simulink model "fft_test"  (Simulink 7.4)
settings: Solver=VariableStepDiscrete  StartTime=0.0  StopTime=500  RelTol=1e-3
libraries: xbsIndex_r4 x1178, casper_library_misc x68, casper_library_delays x13, casper_library_reorder x4, casper_library_ffts_twiddle x2
(part 2 of 11)

== system fft_test/fft/fft_unscrambler ==
  sync : Inport  OutDataType=sfix(16)  OutScaling=2^0
  In1 : Inport  Port=2  OutDataType=sfix(16)  OutScaling=2^0
  In2 : Inport  Port=3  OutDataType=sfix(16)  OutScaling=2^0
  In3 : Inport  Port=4
  In4 : Inport  Port=5
  const : xbsIndex_r4/Constant  arith_type=Boolean  const=1  n_bits=1  bin_pt=0  explicit_period=on  period=1  equ=P=C  opselect=C  inp2=PCIN>>17  opr=+  inp1=P  carry=CIN  dbl_ovrd=off  block_type=constant
      settings: block_version=9.1.01
  reorder : Subsystem  AncestorBlock=casper_library_reorder/reorder  mask(reorder){map=getfield( getfield( get_param( gcb,'UserData' ), 'parameters'),'map'), n_inputs=4, bram_latency=1, map_latency=1, double_buffer=0}
      mask prompts: map "Output Order:"; n_inputs "Number of inputs"; bram_latency "BRAM Latency"; map_latency "Map Latency"; double_buffer "Double Buffer"
      mask init:
      | reorder_init(gcb, ...
      |     'map', map, ...
      |     'n_inputs', n_inputs, ...
      |     'bram_latency', bram_latency, ...
      |     'map_latency', map_latency, ...
      |     'double_buffer', double_buffer);
      settings: AttributesFormatString=order=2
  square_transposer : Subsystem  AncestorBlock=casper_library_reorder/square_transposer  mask(square_transposer){n_inputs=2}
      mask prompts: n_inputs "Number of inputs (2^?):"
      mask init:
      | square_transposer_init(gcb,...
      |     'n_inputs', n_inputs);
      settings: AttributesFormatString=n_inputs=2
  sync_out : Outport  OutDataType=sfix(16)  OutScaling=2^0
  Out1 : Outport  Port=2  OutDataType=sfix(16)  OutScaling=2^0
  Out2 : Outport  Port=3  OutDataType=sfix(16)  OutScaling=2^0
  Out3 : Outport  Port=4
  Out4 : Outport  Port=5
  wires:
  sync/1 -> square_transposer/1(sync)
  square_transposer/1(sync_out) -> reorder/1(sync)
  reorder/1(sync_out) -> sync_out/1
  const/1 -> reorder/2(en)
  In1/1 -> square_transposer/2(In1)
  square_transposer/2(Out1) -> reorder/3(din0)
  reorder/3(dout0) -> Out1/1
  In2/1 -> square_transposer/3(In2)
  square_transposer/3(Out2) -> reorder/4(din1)
  reorder/4(dout1) -> Out2/1
  In3/1 -> square_transposer/4(In3)
  square_transposer/4(Out3) -> reorder/5(din2)
  reorder/5(dout2) -> Out3/1
  In4/1 -> square_transposer/5(In4)
  square_transposer/5(Out4) -> reorder/6(din3)
  reorder/6(dout3) -> Out4/1

== system fft_test/fft/fft_biplex0/biplex_core ==
  pol1 : Inport
  pol2 : Inport  Port=2
  sync : Inport  Port=3
  shift : Inport  Port=4
  Constant : xbsIndex_r4/Constant  arith_type=Boolean  const=0  n_bits=16  bin_pt=14  explicit_period=off  period=1  equ=P=C  opselect=C  inp2=PCIN>>17  opr=+  inp1=P  carry=CIN  dbl_ovrd=off  block_type=constant
      settings: block_version=11.4
  fft_stage_1 : Subsystem  AncestorBlock=casper_library_ffts/fft_stage_n  mask(fft_stage_n){FFTSize=4, FFTStage=1, input_bit_width=8, coeff_bit_width=8, delays_bram=off, coeffs_bram=off, quantization=Round  (unbiased: +/- Inf), overflow=Saturate, add_latency=2, mult_latency=3, bram_latency=1, conv_latency=2, arch=Virtex5, opt_target=multipliers, use_hdl=on, use_embedded=off, dsp48_adders=on}
      mask prompts: FFTSize "Size of FFT: (2^? pnts)"; FFTStage "Stage of FFT:"; input_bit_width "Input/Output Bit Width:"; coeff_bit_width "Coefficient Bit Width"; delays_bram "Implement Delays in BRAM:"; coeffs_bram "Store Coefficients in BRAM:"; quantization "Quantization Behavior"; overflow "Overflow Behavior"; add_latency "Add Latency"; mult_latency "Mult Latency"; bram_latency "BRAM Latency"; conv_latency "Convert latency"; arch "Architecture"; opt_target "Use less"; use_hdl "Use behavioural HDL for mutlipliers"; use_embedded "Use embedded multipliers"; dsp48_adders "Use DSP48s for adders"
      mask init:
      | fft_stage_n_init(gcb,...
      |     'FFTSize', FFTSize,...
      |     'FFTStage', FFTStage,...
      |     'input_bit_width', input_bit_width,...
      |     'coeff_bit_width', coeff_bit_width,...
      |     'delays_bram', delays_bram,...
      |     'coeffs_bram', coeffs_bram,...
      |     'quantization', quantization,...
      |     'overflow', overflow,...
      |     'add_latency', add_latency,...
      |     'mult_latency', mult_latency,...
      |     'bram_latency', bram_latency,...
      |     'conv_latency', conv_latency, ...
      |     'arch', arch, ...
      |     'opt_target', opt_target, ...
      |     'use_hdl', use_hdl,...
      |     'use_embedded', use_embedded, ...
      |     'dsp48_adders', dsp48_adders);
      settings: AttributesFormatString=|
      | [1/4]
      | delays in slices
      | coeffs in slices
      mask StyleString: edit,edit,edit,edit,checkbox,checkbox,popup(Truncate|Round  (unbiased: +/- Inf)|Round  (unbiased: Even Values)),popup(Wrap|Saturate|Error),edit,edit,edit,edit,popup(Virtex2Pro|Virtex5),popup(logic|multipliers),checkbox,checkbox,checkbox
      mask CallbackString:
      | ||||||||||||fft_callback_arch(gcb);||use_hdl = get_param(gcb,'use_hdl');
      | visibs = get_param(gcb, 'MaskVisibilities');
      | if( strcmp(use_hdl,'on')),
      |     visibs{16} = 'off';
      | else,
      |     visibs{16} = 'on';
      | end
      |     set_param(gcb, 'MaskVisibilities',visibs);||fft_callback_dsp48_adders(gcb);
  fft_stage_2 : Subsystem  AncestorBlock=casper_library_ffts/fft_stage_n  mask(fft_stage_n){FFTSize=4, FFTStage=2, input_bit_width=8, coeff_bit_width=8, delays_bram=off, coeffs_bram=off, quantization=Round  (unbiased: +/- Inf), overflow=Saturate, add_latency=2, mult_latency=3, bram_latency=1, conv_latency=2, arch=Virtex5, opt_target=multipliers, use_hdl=off, use_embedded=on, dsp48_adders=on}
      mask prompts: FFTSize "Size of FFT: (2^? pnts)"; FFTStage "Stage of FFT:"; input_bit_width "Input/Output Bit Width:"; coeff_bit_width "Coefficient Bit Width"; delays_bram "Implement Delays in BRAM:"; coeffs_bram "Store Coefficients in BRAM:"; quantization "Quantization Behavior"; overflow "Overflow Behavior"; add_latency "Add Latency"; mult_latency "Mult Latency"; bram_latency "BRAM Latency"; conv_latency "Convert latency"; arch "Architecture"; opt_target "Use less"; use_hdl "Use behavioural HDL for mutlipliers"; use_embedded "Use embedded multipliers"; dsp48_adders "Use DSP48s for adders"
      mask init: same as fft_test/fft/fft_biplex0/biplex_core/fft_stage_1
      settings: AttributesFormatString=|
      | [2/4]
      | delays in slices
      | coeffs in slices
      mask StyleString: edit,edit,edit,edit,checkbox,checkbox,popup(Truncate|Round  (unbiased: +/- Inf)|Round  (unbiased: Even Values)),popup(Wrap|Saturate|Error),edit,edit,edit,edit,popup(Virtex2Pro|Virtex5),popup(logic|multipliers),checkbox,checkbox,checkbox
      mask CallbackString:
      | ||||||||||||fft_callback_arch(gcb);||use_hdl = get_param(gcb,'use_hdl');
      | visibs = get_param(gcb, 'MaskVisibilities');
      | if( strcmp(use_hdl,'on')),
      |     visibs{16} = 'off';
      | else,
      |     visibs{16} = 'on';
      | end
      |     set_param(gcb, 'MaskVisibilities',visibs);||fft_callback_dsp48_adders(gcb);
  fft_stage_3 : Subsystem  AncestorBlock=casper_library_ffts/fft_stage_n  mask(fft_stage_n){FFTSize=4, FFTStage=3, input_bit_width=8, coeff_bit_width=8, delays_bram=off, coeffs_bram=off, quantization=Round  (unbiased: +/- Inf), overflow=Saturate, add_latency=2, mult_latency=3, bram_latency=1, conv_latency=2, arch=Virtex5, opt_target=multipliers, use_hdl=on, use_embedded=off, dsp48_adders=on}
      mask prompts: FFTSize "Size of FFT: (2^? pnts)"; FFTStage "Stage of FFT:"; input_bit_width "Input/Output Bit Width:"; coeff_bit_width "Coefficient Bit Width"; delays_bram "Implement Delays in BRAM:"; coeffs_bram "Store Coefficients in BRAM:"; quantization "Quantization Behavior"; overflow "Overflow Behavior"; add_latency "Add Latency"; mult_latency "Mult Latency"; bram_latency "BRAM Latency"; conv_latency "Convert latency"; arch "Architecture"; opt_target "Use less"; use_hdl "Use behavioural HDL for mutlipliers"; use_embedded "Use embedded multipliers"; dsp48_adders "Use DSP48s for adders"
      mask init: same as fft_test/fft/fft_biplex0/biplex_core/fft_stage_1
      settings: AttributesFormatString=|
      | [3/4]
      | delays in slices
      | coeffs in slices
      mask StyleString: edit,edit,edit,edit,checkbox,checkbox,popup(Truncate|Round  (unbiased: +/- Inf)|Round  (unbiased: Even Values)),popup(Wrap|Saturate|Error),edit,edit,edit,edit,popup(Virtex2Pro|Virtex5),popup(logic|multipliers),checkbox,checkbox,checkbox
      mask CallbackString:
      | ||||||||||||fft_callback_arch(gcb);||use_hdl = get_param(gcb,'use_hdl');
      | visibs = get_param(gcb, 'MaskVisibilities');
      | if( strcmp(use_hdl,'on')),
      |     visibs{16} = 'off';
      | else,
      |     visibs{16} = 'on';
      | end
      |     set_param(gcb, 'MaskVisibilities',visibs);||fft_callback_dsp48_adders(gcb);
  fft_stage_4 : Subsystem  AncestorBlock=casper_library_ffts/fft_stage_n  mask(fft_stage_n){FFTSize=4, FFTStage=4, input_bit_width=8, coeff_bit_width=8, delays_bram=off, coeffs_bram=off, quantization=Round  (unbiased: +/- Inf), overflow=Saturate, add_latency=2, mult_latency=3, bram_latency=1, conv_latency=2, arch=Virtex5, opt_target=multipliers, use_hdl=on, use_embedded=off, dsp48_adders=on}
      mask prompts: FFTSize "Size of FFT: (2^? pnts)"; FFTStage "Stage of FFT:"; input_bit_width "Input/Output Bit Width:"; coeff_bit_width "Coefficient Bit Width"; delays_bram "Implement Delays in BRAM:"; coeffs_bram "Store Coefficients in BRAM:"; quantization "Quantization Behavior"; overflow "Overflow Behavior"; add_latency "Add Latency"; mult_latency "Mult Latency"; bram_latency "BRAM Latency"; conv_latency "Convert latency"; arch "Architecture"; opt_target "Use less"; use_hdl "Use behavioural HDL for mutlipliers"; use_embedded "Use embedded multipliers"; dsp48_adders "Use DSP48s for adders"
      mask init: same as fft_test/fft/fft_biplex0/biplex_core/fft_stage_1
      settings: AttributesFormatString=|
      | [4/4]
      | delays in slices
      | coeffs in slices
      mask StyleString: edit,edit,edit,edit,checkbox,checkbox,popup(Truncate|Round  (unbiased: +/- Inf)|Round  (unbiased: Even Values)),popup(Wrap|Saturate|Error),edit,edit,edit,edit,popup(Virtex2Pro|Virtex5),popup(logic|multipliers),checkbox,checkbox,checkbox
      mask CallbackString:
      | ||||||||||||fft_callback_arch(gcb);||use_hdl = get_param(gcb,'use_hdl');
      | visibs = get_param(gcb, 'MaskVisibilities');
      | if( strcmp(use_hdl,'on')),
      |     visibs{16} = 'off';
      | else,
      |     visibs{16} = 'on';
      | end
      |     set_param(gcb, 'MaskVisibilities',visibs);||fft_callback_dsp48_adders(gcb);
  out1 : Outport
  out2 : Outport  Port=2
  of : Outport  Port=3
  sync_out : Outport  Port=4
  wires:
  fft_stage_1/1(out1) -> fft_stage_2/1(in1)
  fft_stage_1/2(out2) -> fft_stage_2/2(in2)
  fft_stage_1/3(of) -> fft_stage_2/3(of_in)
  fft_stage_1/4(sync_out) -> fft_stage_2/4(sync)
  shift/1 -> fft_stage_2/5(shift), fft_stage_3/5(shift), fft_stage_4/5(shift), fft_stage_1/5(shift)
  fft_stage_2/1(out1) -> fft_stage_3/1(in1)
  fft_stage_2/2(out2) -> fft_stage_3/2(in2)
  fft_stage_2/3(of) -> fft_stage_3/3(of_in)
  fft_stage_2/4(sync_out) -> fft_stage_3/4(sync)
  fft_stage_3/1(out1) -> fft_stage_4/1(in1)
  fft_stage_3/2(out2) -> fft_stage_4/2(in2)
  fft_stage_3/3(of) -> fft_stage_4/3(of_in)
  fft_stage_3/4(sync_out) -> fft_stage_4/4(sync)
  pol1/1 -> fft_stage_1/1(in1)
  pol2/1 -> fft_stage_1/2(in2)
  Constant/1 -> fft_stage_1/3(of_in)
  sync/1 -> fft_stage_1/4(sync)
  fft_stage_4/1(out1) -> out1/1
  fft_stage_4/2(out2) -> out2/1
  fft_stage_4/3(of) -> of/1
  fft_stage_4/4(sync_out) -> sync_out/1

== system fft_test/fft/fft_biplex0/biplex_cplx_unscrambler ==
  even : Inport  OutDataType=sfix(16)  OutScaling=2^0
  odd : Inport  Port=2  OutDataType=sfix(16)  OutScaling=2^0
  sync : Inport  Port=3  OutDataType=sfix(16)  OutScaling=2^0
  Constant : xbsIndex_r4/Constant  arith_type=Boolean  const=1  n_bits=1  bin_pt=0  explicit_period=on  period=1  equ=P=C  opselect=C  inp2=PCIN>>17  opr=+  inp1=P  carry=CIN  dbl_ovrd=off  block_type=constant
      settings: block_version=9.1.01
  Constant1 : xbsIndex_r4/Constant  arith_type=Unsigned  const=2^(FFTSize-1)  n_bits=FFTSize  bin_pt=0  explicit_period=on  period=1  equ=P=C  opselect=C  inp2=PCIN>>17  opr=+  inp1=P  carry=CIN  dbl_ovrd=off  block_type=constant
      settings: block_version=9.1.01
  Constant2 : xbsIndex_r4/Constant  arith_type=Unsigned  const=2^(FFTSize-1)  n_bits=FFTSize  bin_pt=0  explicit_period=on  period=1  equ=P=C  opselect=C  inp2=PCIN>>17  opr=+  inp1=P  carry=CIN  dbl_ovrd=off  block_type=constant
      settings: block_version=9.1.01
  Convert : xbsIndex_r4/Convert  arith_type=Unsigned  n_bits=1  bin_pt=0  quantization=Truncate  overflow=Wrap  latency=0  dbl_ovrd=off  pipeline=off  block_type=convert
      settings: xl_area=[0, 0, 0, 0, 0, 0, 0]
  Convert1 : xbsIndex_r4/Convert  arith_type=Unsigned  n_bits=1  bin_pt=0  quantization=Truncate  overflow=Wrap  latency=0  dbl_ovrd=off  pipeline=off  block_type=convert
      settings: xl_area=[0, 0, 0, 0, 0, 0, 0]
  Counter : xbsIndex_r4/Counter  cnt_type=Free Running  cnt_to=Inf  operation=Up  start_count=0  cnt_by_val=1  arith_type=Unsigned  n_bits=FFTSize  bin_pt=0  load_pin=off  rst=on  en=off  explicit_period=off  period=1  dbl_ovrd=off  use_behavioral_HDL=off  implementation=Fabric  use_rpm=on  block_type=counter
      settings: xl_area=[0, 0, 0, 0, 0, 0, 0]  block_version=9.1.01
  Counter1 : xbsIndex_r4/Counter  cnt_type=Free Running  cnt_to=Inf  operation=Up  start_count=0  cnt_by_val=1  arith_type=Unsigned  n_bits=FFTSize  bin_pt=0  load_pin=off  rst=on  en=off  explicit_period=off  period=1  dbl_ovrd=off  use_behavioral_HDL=off  implementation=Fabric  use_rpm=on  block_type=counter
      settings: xl_area=[0, 0, 0, 0, 0, 0, 0]  block_version=9.1.01
  Relational : xbsIndex_r4/Relational  mode=a<=b  en=off  latency=0  dbl_ovrd=off  block_type=relational
      settings: xl_area=[0, 0, 0, 0, 0, 0, 0]  block_version=9.1.01
  Relational1 : xbsIndex_r4/Relational  mode=a<=b  en=off  latency=0  dbl_ovrd=off  block_type=relational
      settings: xl_area=[0, 0, 0, 0, 0, 0, 0]  block_version=9.1.01
  barrel_switcher : casper_library_reorder/barrel_switcher  SystemSampleTime=-1  n_inputs=1
      settings: AttributesFormatString=n_inputs=1
  barrel_switcher1 : casper_library_reorder/barrel_switcher  SystemSampleTime=-1  n_inputs=1
      settings: AttributesFormatString=n_inputs=1
  reorder : Subsystem  AncestorBlock=casper_library_reorder/reorder  mask(reorder){map=getfield( getfield( get_param( gcb,'UserData' ), 'parameters'),'map'), n_inputs=1, bram_latency=1, map_latency=0, double_buffer=0, bram_map=off}
      mask prompts: map "Output Order:"; n_inputs "Number of inputs"; bram_latency "BRAM Latency"; map_latency "Map Latency"; double_buffer "Double Buffer"; bram_map "Use BlockRAM for Map"
      mask init:
      | reorder_init(gcb, ...
      |     'map', map, ...
      |     'n_inputs', n_inputs, ...
      |     'bram_latency', bram_latency, ...
      |     'map_latency', map_latency, ...
      |     'double_buffer', double_buffer, ...
      |     'bram_map', bram_map);
      settings: AttributesFormatString=order=2
      mask Help: eval('xlWeb(''http://casper.berkeley.edu/wiki/Reorder'')')
  reorder1 : Subsystem  AncestorBlock=casper_library_reorder/reorder  mask(reorder){map=getfield( getfield( get_param( gcb,'UserData' ), 'parameters'),'map'), n_inputs=1, bram_latency=1, map_latency=0, double_buffer=0, bram_map=off}
      mask prompts: map "Output Order:"; n_inputs "Number of inputs"; bram_latency "BRAM Latency"; map_latency "Map Latency"; double_buffer "Double Buffer"; bram_map "Use BlockRAM for Map"
      mask init: same as fft_test/fft/fft_biplex0/biplex_cplx_unscrambler/reorder
      settings: AttributesFormatString=order=2
      mask Help: eval('xlWeb(''http://casper.berkeley.edu/wiki/Reorder'')')
  pol1 : Outport  OutDataType=sfix(16)  OutScaling=2^0
  pol2 : Outport  Port=2  OutDataType=sfix(16)  OutScaling=2^0
  sync_out : Outport  Port=3  OutDataType=sfix(16)  OutScaling=2^0
  wires:
  barrel_switcher/1 -> reorder/1(sync), reorder1/1(sync)
  barrel_switcher/2 -> reorder/3(din0)
  barrel_switcher/3 -> reorder1/3(din0)
  reorder/1(sync_out) -> barrel_switcher1/2, Counter1/1
  reorder/3(dout0) -> barrel_switcher1/3
  reorder1/3(dout0) -> barrel_switcher1/4
  even/1 -> barrel_switcher/3
  odd/1 -> barrel_switcher/4
  barrel_switcher1/1 -> sync_out/1
  barrel_switcher1/2 -> pol1/1
  barrel_switcher1/3 -> pol2/1
  sync/1 -> barrel_switcher/2, Counter/1
  Constant/1 -> reorder/2(en), reorder1/2(en)
  Constant1/1 -> Relational/1
  Counter/1 -> Relational/2
  Counter1/1 -> Relational1/2
  Constant2/1 -> Relational1/1
  Relational/1 -> Convert/1
  Relational1/1 -> Convert1/1
  Convert1/1 -> barrel_switcher1/1
  Convert/1 -> barrel_switcher/1

== system fft_test/fft/fft_biplex1/biplex_core ==
  pol1 : Inport
  pol2 : Inport  Port=2
  sync : Inport  Port=3
  shift : Inport  Port=4
  Constant : xbsIndex_r4/Constant  arith_type=Boolean  const=0  n_bits=16  bin_pt=14  explicit_period=off  period=1  equ=P=C  opselect=C  inp2=PCIN>>17  opr=+  inp1=P  carry=CIN  dbl_ovrd=off  block_type=constant
      settings: block_version=11.4
  fft_stage_1 : Subsystem  AncestorBlock=casper_library_ffts/fft_stage_n  mask(fft_stage_n){FFTSize=4, FFTStage=1, input_bit_width=8, coeff_bit_width=8, delays_bram=off, coeffs_bram=off, quantization=Round  (unbiased: +/- Inf), overflow=Saturate, add_latency=2, mult_latency=3, bram_latency=1, conv_latency=2, arch=Virtex5, opt_target=multipliers, use_hdl=on, use_embedded=off, dsp48_adders=on}
      mask prompts: FFTSize "Size of FFT: (2^? pnts)"; FFTStage "Stage of FFT:"; input_bit_width "Input/Output Bit Width:"; coeff_bit_width "Coefficient Bit Width"; delays_bram "Implement Delays in BRAM:"; coeffs_bram "Store Coefficients in BRAM:"; quantization "Quantization Behavior"; overflow "Overflow Behavior"; add_latency "Add Latency"; mult_latency "Mult Latency"; bram_latency "BRAM Latency"; conv_latency "Convert latency"; arch "Architecture"; opt_target "Use less"; use_hdl "Use behavioural HDL for mutlipliers"; use_embedded "Use embedded multipliers"; dsp48_adders "Use DSP48s for adders"
      mask init: same as fft_test/fft/fft_biplex0/biplex_core/fft_stage_1
      settings: AttributesFormatString=|
      | [1/4]
      | delays in slices
      | coeffs in slices
      mask StyleString: edit,edit,edit,edit,checkbox,checkbox,popup(Truncate|Round  (unbiased: +/- Inf)|Round  (unbiased: Even Values)),popup(Wrap|Saturate|Error),edit,edit,edit,edit,popup(Virtex2Pro|Virtex5),popup(logic|multipliers),checkbox,checkbox,checkbox
      mask CallbackString:
      | ||||||||||||fft_callback_arch(gcb);||use_hdl = get_param(gcb,'use_hdl');
      | visibs = get_param(gcb, 'MaskVisibilities');
      | if( strcmp(use_hdl,'on')),
      |     visibs{16} = 'off';
      | else,
      |     visibs{16} = 'on';
      | end
      |     set_param(gcb, 'MaskVisibilities',visibs);||fft_callback_dsp48_adders(gcb);
  fft_stage_2 : Subsystem  AncestorBlock=casper_library_ffts/fft_stage_n  mask(fft_stage_n){FFTSize=4, FFTStage=2, input_bit_width=8, coeff_bit_width=8, delays_bram=off, coeffs_bram=off, quantization=Round  (unbiased: +/- Inf), overflow=Saturate, add_latency=2, mult_latency=3, bram_latency=1, conv_latency=2, arch=Virtex5, opt_target=multipliers, use_hdl=off, use_embedded=on, dsp48_adders=on}
      mask prompts: FFTSize "Size of FFT: (2^? pnts)"; FFTStage "Stage of FFT:"; input_bit_width "Input/Output Bit Width:"; coeff_bit_width "Coefficient Bit Width"; delays_bram "Implement Delays in BRAM:"; coeffs_bram "Store Coefficients in BRAM:"; quantization "Quantization Behavior"; overflow "Overflow Behavior"; add_latency "Add Latency"; mult_latency "Mult Latency"; bram_latency "BRAM Latency"; conv_latency "Convert latency"; arch "Architecture"; opt_target "Use less"; use_hdl "Use behavioural HDL for mutlipliers"; use_embedded "Use embedded multipliers"; dsp48_adders "Use DSP48s for adders"
      mask init: same as fft_test/fft/fft_biplex0/biplex_core/fft_stage_1
      settings: AttributesFormatString=|
      | [2/4]
      | delays in slices
      | coeffs in slices
      mask StyleString: edit,edit,edit,edit,checkbox,checkbox,popup(Truncate|Round  (unbiased: +/- Inf)|Round  (unbiased: Even Values)),popup(Wrap|Saturate|Error),edit,edit,edit,edit,popup(Virtex2Pro|Virtex5),popup(logic|multipliers),checkbox,checkbox,checkbox
      mask CallbackString:
      | ||||||||||||fft_callback_arch(gcb);||use_hdl = get_param(gcb,'use_hdl');
      | visibs = get_param(gcb, 'MaskVisibilities');
      | if( strcmp(use_hdl,'on')),
      |     visibs{16} = 'off';
      | else,
      |     visibs{16} = 'on';
      | end
      |     set_param(gcb, 'MaskVisibilities',visibs);||fft_callback_dsp48_adders(gcb);
  fft_stage_3 : Subsystem  AncestorBlock=casper_library_ffts/fft_stage_n  mask(fft_stage_n){FFTSize=4, FFTStage=3, input_bit_width=8, coeff_bit_width=8, delays_bram=off, coeffs_bram=off, quantization=Round  (unbiased: +/- Inf), overflow=Saturate, add_latency=2, mult_latency=3, bram_latency=1, conv_latency=2, arch=Virtex5, opt_target=multipliers, use_hdl=on, use_embedded=off, dsp48_adders=on}
      mask prompts: FFTSize "Size of FFT: (2^? pnts)"; FFTStage "Stage of FFT:"; input_bit_width "Input/Output Bit Width:"; coeff_bit_width "Coefficient Bit Width"; delays_bram "Implement Delays in BRAM:"; coeffs_bram "Store Coefficients in BRAM:"; quantization "Quantization Behavior"; overflow "Overflow Behavior"; add_latency "Add Latency"; mult_latency "Mult Latency"; bram_latency "BRAM Latency"; conv_latency "Convert latency"; arch "Architecture"; opt_target "Use less"; use_hdl "Use behavioural HDL for mutlipliers"; use_embedded "Use embedded multipliers"; dsp48_adders "Use DSP48s for adders"
      mask init: same as fft_test/fft/fft_biplex0/biplex_core/fft_stage_1
      settings: AttributesFormatString=|
      | [3/4]
      | delays in slices
      | coeffs in slices
      mask StyleString: edit,edit,edit,edit,checkbox,checkbox,popup(Truncate|Round  (unbiased: +/- Inf)|Round  (unbiased: Even Values)),popup(Wrap|Saturate|Error),edit,edit,edit,edit,popup(Virtex2Pro|Virtex5),popup(logic|multipliers),checkbox,checkbox,checkbox
      mask CallbackString:
      | ||||||||||||fft_callback_arch(gcb);||use_hdl = get_param(gcb,'use_hdl');
      | visibs = get_param(gcb, 'MaskVisibilities');
      | if( strcmp(use_hdl,'on')),
      |     visibs{16} = 'off';
      | else,
      |     visibs{16} = 'on';
      | end
      |     set_param(gcb, 'MaskVisibilities',visibs);||fft_callback_dsp48_adders(gcb);
  fft_stage_4 : Subsystem  AncestorBlock=casper_library_ffts/fft_stage_n  mask(fft_stage_n){FFTSize=4, FFTStage=4, input_bit_width=8, coeff_bit_width=8, delays_bram=off, coeffs_bram=off, quantization=Round  (unbiased: +/- Inf), overflow=Saturate, add_latency=2, mult_latency=3, bram_latency=1, conv_latency=2, arch=Virtex5, opt_target=multipliers, use_hdl=on, use_embedded=off, dsp48_adders=on}
      mask prompts: FFTSize "Size of FFT: (2^? pnts)"; FFTStage "Stage of FFT:"; input_bit_width "Input/Output Bit Width:"; coeff_bit_width "Coefficient Bit Width"; delays_bram "Implement Delays in BRAM:"; coeffs_bram "Store Coefficients in BRAM:"; quantization "Quantization Behavior"; overflow "Overflow Behavior"; add_latency "Add Latency"; mult_latency "Mult Latency"; bram_latency "BRAM Latency"; conv_latency "Convert latency"; arch "Architecture"; opt_target "Use less"; use_hdl "Use behavioural HDL for mutlipliers"; use_embedded "Use embedded multipliers"; dsp48_adders "Use DSP48s for adders"
      mask init: same as fft_test/fft/fft_biplex0/biplex_core/fft_stage_1
      settings: AttributesFormatString=|
      | [4/4]
      | delays in slices
      | coeffs in slices
      mask StyleString: edit,edit,edit,edit,checkbox,checkbox,popup(Truncate|Round  (unbiased: +/- Inf)|Round  (unbiased: Even Values)),popup(Wrap|Saturate|Error),edit,edit,edit,edit,popup(Virtex2Pro|Virtex5),popup(logic|multipliers),checkbox,checkbox,checkbox
      mask CallbackString:
      | ||||||||||||fft_callback_arch(gcb);||use_hdl = get_param(gcb,'use_hdl');
      | visibs = get_param(gcb, 'MaskVisibilities');
      | if( strcmp(use_hdl,'on')),
      |     visibs{16} = 'off';
      | else,
      |     visibs{16} = 'on';
      | end
      |     set_param(gcb, 'MaskVisibilities',visibs);||fft_callback_dsp48_adders(gcb);
  out1 : Outport
  out2 : Outport  Port=2
  of : Outport  Port=3
  sync_out : Outport  Port=4
  wires:
  fft_stage_1/1(out1) -> fft_stage_2/1(in1)
  fft_stage_1/2(out2) -> fft_stage_2/2(in2)
  fft_stage_1/3(of) -> fft_stage_2/3(of_in)
  fft_stage_1/4(sync_out) -> fft_stage_2/4(sync)
  shift/1 -> fft_stage_2/5(shift), fft_stage_3/5(shift), fft_stage_4/5(shift), fft_stage_1/5(shift)
  fft_stage_2/1(out1) -> fft_stage_3/1(in1)
  fft_stage_2/2(out2) -> fft_stage_3/2(in2)
  fft_stage_2/3(of) -> fft_stage_3/3(of_in)
  fft_stage_2/4(sync_out) -> fft_stage_3/4(sync)
  fft_stage_3/1(out1) -> fft_stage_4/1(in1)
  fft_stage_3/2(out2) -> fft_stage_4/2(in2)
  fft_stage_3/3(of) -> fft_stage_4/3(of_in)
  fft_stage_3/4(sync_out) -> fft_stage_4/4(sync)
  pol1/1 -> fft_stage_1/1(in1)
  pol2/1 -> fft_stage_1/2(in2)
  Constant/1 -> fft_stage_1/3(of_in)
  sync/1 -> fft_stage_1/4(sync)
  fft_stage_4/1(out1) -> out1/1
  fft_stage_4/2(out2) -> out2/1
  fft_stage_4/3(of) -> of/1
  fft_stage_4/4(sync_out) -> sync_out/1

== system fft_test/fft/fft_biplex1/biplex_cplx_unscrambler ==
  even : Inport  OutDataType=sfix(16)  OutScaling=2^0
  odd : Inport  Port=2  OutDataType=sfix(16)  OutScaling=2^0
  sync : Inport  Port=3  OutDataType=sfix(16)  OutScaling=2^0
  Constant : xbsIndex_r4/Constant  arith_type=Boolean  const=1  n_bits=1  bin_pt=0  explicit_period=on  period=1  equ=P=C  opselect=C  inp2=PCIN>>17  opr=+  inp1=P  carry=CIN  dbl_ovrd=off  block_type=constant
      settings: block_version=9.1.01
  Constant1 : xbsIndex_r4/Constant  arith_type=Unsigned  const=2^(FFTSize-1)  n_bits=FFTSize  bin_pt=0  explicit_period=on  period=1  equ=P=C  opselect=C  inp2=PCIN>>17  opr=+  inp1=P  carry=CIN  dbl_ovrd=off  block_type=constant
      settings: block_version=9.1.01
  Constant2 : xbsIndex_r4/Constant  arith_type=Unsigned  const=2^(FFTSize-1)  n_bits=FFTSize  bin_pt=0  explicit_period=on  period=1  equ=P=C  opselect=C  inp2=PCIN>>17  opr=+  inp1=P  carry=CIN  dbl_ovrd=off  block_type=constant
      settings: block_version=9.1.01
  Convert : xbsIndex_r4/Convert  arith_type=Unsigned  n_bits=1  bin_pt=0  quantization=Truncate  overflow=Wrap  latency=0  dbl_ovrd=off  pipeline=off  block_type=convert
      settings: xl_area=[0, 0, 0, 0, 0, 0, 0]
  Convert1 : xbsIndex_r4/Convert  arith_type=Unsigned  n_bits=1  bin_pt=0  quantization=Truncate  overflow=Wrap  latency=0  dbl_ovrd=off  pipeline=off  block_type=convert
      settings: xl_area=[0, 0, 0, 0, 0, 0, 0]
  Counter : xbsIndex_r4/Counter  cnt_type=Free Running  cnt_to=Inf  operation=Up  start_count=0  cnt_by_val=1  arith_type=Unsigned  n_bits=FFTSize  bin_pt=0  load_pin=off  rst=on  en=off  explicit_period=off  period=1  dbl_ovrd=off  use_behavioral_HDL=off  implementation=Fabric  use_rpm=on  block_type=counter
      settings: xl_area=[0, 0, 0, 0, 0, 0, 0]  block_version=9.1.01
  Counter1 : xbsIndex_r4/Counter  cnt_type=Free Running  cnt_to=Inf  operation=Up  start_count=0  cnt_by_val=1  arith_type=Unsigned  n_bits=FFTSize  bin_pt=0  load_pin=off  rst=on  en=off  explicit_period=off  period=1  dbl_ovrd=off  use_behavioral_HDL=off  implementation=Fabric  use_rpm=on  block_type=counter
      settings: xl_area=[0, 0, 0, 0, 0, 0, 0]  block_version=9.1.01
  Relational : xbsIndex_r4/Relational  mode=a<=b  en=off  latency=0  dbl_ovrd=off  block_type=relational
      settings: xl_area=[0, 0, 0, 0, 0, 0, 0]  block_version=9.1.01
  Relational1 : xbsIndex_r4/Relational  mode=a<=b  en=off  latency=0  dbl_ovrd=off  block_type=relational
      settings: xl_area=[0, 0, 0, 0, 0, 0, 0]  block_version=9.1.01
  barrel_switcher : casper_library_reorder/barrel_switcher  SystemSampleTime=-1  n_inputs=1
      settings: AttributesFormatString=n_inputs=1
  barrel_switcher1 : casper_library_reorder/barrel_switcher  SystemSampleTime=-1  n_inputs=1
      settings: AttributesFormatString=n_inputs=1
  reorder : Subsystem  AncestorBlock=casper_library_reorder/reorder  mask(reorder){map=getfield( getfield( get_param( gcb,'UserData' ), 'parameters'),'map'), n_inputs=1, bram_latency=1, map_latency=0, double_buffer=0, bram_map=off}
      mask prompts: map "Output Order:"; n_inputs "Number of inputs"; bram_latency "BRAM Latency"; map_latency "Map Latency"; double_buffer "Double Buffer"; bram_map "Use BlockRAM for Map"
      mask init: same as fft_test/fft/fft_biplex0/biplex_cplx_unscrambler/reorder
      settings: AttributesFormatString=order=2
      mask Help: eval('xlWeb(''http://casper.berkeley.edu/wiki/Reorder'')')
  reorder1 : Subsystem  AncestorBlock=casper_library_reorder/reorder  mask(reorder){map=getfield( getfield( get_param( gcb,'UserData' ), 'parameters'),'map'), n_inputs=1, bram_latency=1, map_latency=0, double_buffer=0, bram_map=off}
      mask prompts: map "Output Order:"; n_inputs "Number of inputs"; bram_latency "BRAM Latency"; map_latency "Map Latency"; double_buffer "Double Buffer"; bram_map "Use BlockRAM for Map"
      mask init: same as fft_test/fft/fft_biplex0/biplex_cplx_unscrambler/reorder
      settings: AttributesFormatString=order=2
      mask Help: eval('xlWeb(''http://casper.berkeley.edu/wiki/Reorder'')')
  pol1 : Outport  OutDataType=sfix(16)  OutScaling=2^0
  pol2 : Outport  Port=2  OutDataType=sfix(16)  OutScaling=2^0
  sync_out : Outport  Port=3  OutDataType=sfix(16)  OutScaling=2^0
  wires:
  barrel_switcher/1 -> reorder/1(sync), reorder1/1(sync)
  barrel_switcher/2 -> reorder/3(din0)
  barrel_switcher/3 -> reorder1/3(din0)
  reorder/1(sync_out) -> barrel_switcher1/2, Counter1/1
  reorder/3(dout0) -> barrel_switcher1/3
  reorder1/3(dout0) -> barrel_switcher1/4
  even/1 -> barrel_switcher/3
  odd/1 -> barrel_switcher/4
  barrel_switcher1/1 -> sync_out/1
  barrel_switcher1/2 -> pol1/1
  barrel_switcher1/3 -> pol2/1
  sync/1 -> barrel_switcher/2, Counter/1
  Constant/1 -> reorder/2(en), reorder1/2(en)
  Constant1/1 -> Relational/1
  Counter/1 -> Relational/2
  Counter1/1 -> Relational1/2
  Constant2/1 -> Relational1/1
  Relational/1 -> Convert/1
  Relational1/1 -> Convert1/1
  Convert1/1 -> barrel_switcher1/1
  Convert/1 -> barrel_switcher/1

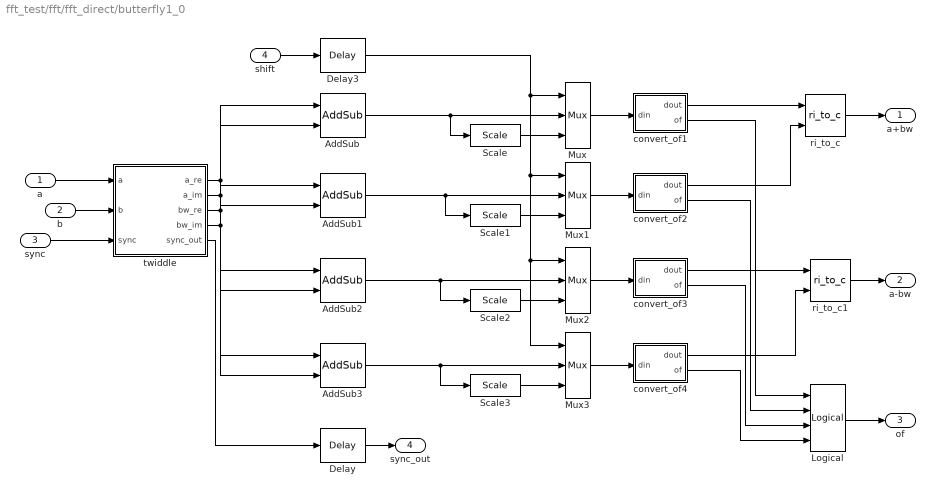
== system fft_test/fft/fft_direct/butterfly1_0 ==
  a : Inport  OutDataType=sfix(16)  OutScaling=2^0
  b : Inport  Port=2  OutDataType=sfix(16)  OutScaling=2^0
  sync : Inport  Port=3  OutDataType=sfix(16)  OutScaling=2^0
  shift : Inport  Port=4  OutDataType=sfix(16)  OutScaling=2^0
  AddSub : xbsIndex_r4/AddSub  mode=Addition  use_carryin=off  use_carryout=off  en=off  latency=add_latency  precision=Full  arith_type=Unsigned  n_bits=8  bin_pt=2  quantization=Truncate  overflow=Wrap  dbl_ovrd=off  use_behavioral_HDL=off  hw_selection=DSP48  pipelined=on  use_rpm=on  block_type=addsub
      settings: xl_area=[0, 0, 0, 0, 0, 0, 0]  block_version=9.1.01
  AddSub1 : xbsIndex_r4/AddSub  mode=Addition  use_carryin=off  use_carryout=off  en=off  latency=add_latency  precision=Full  arith_type=Unsigned  n_bits=8  bin_pt=2  quantization=Truncate  overflow=Wrap  dbl_ovrd=off  use_behavioral_HDL=off  hw_selection=DSP48  pipelined=on  use_rpm=on  block_type=addsub
      settings: xl_area=[0, 0, 0, 0, 0, 0, 0]  block_version=9.1.01
  AddSub2 : xbsIndex_r4/AddSub  mode=Subtraction  use_carryin=off  use_carryout=off  en=off  latency=add_latency  precision=Full  arith_type=Unsigned  n_bits=8  bin_pt=2  quantization=Truncate  overflow=Wrap  dbl_ovrd=off  use_behavioral_HDL=off  hw_selection=DSP48  pipelined=on  use_rpm=on  block_type=addsub
      settings: xl_area=[0, 0, 0, 0, 0, 0, 0]  block_version=9.1.01
  AddSub3 : xbsIndex_r4/AddSub  mode=Subtraction  use_carryin=off  use_carryout=off  en=off  latency=add_latency  precision=Full  arith_type=Unsigned  n_bits=8  bin_pt=2  quantization=Truncate  overflow=Wrap  dbl_ovrd=off  use_behavioral_HDL=off  hw_selection=DSP48  pipelined=on  use_rpm=on  block_type=addsub
      settings: xl_area=[0, 0, 0, 0, 0, 0, 0]  block_version=9.1.01
  Delay : xbsIndex_r4/Delay  en=off  latency=add_latency + conv_latency + 1  dbl_ovrd=off  reg_retiming=on  block_type=delay
      settings: xl_area=[0, 0, 0, 0, 0, 0, 0]  block_version=9.1.01
  Delay3 : xbsIndex_r4/Delay  en=off  latency=add_latency  dbl_ovrd=off  reg_retiming=off  block_type=delay
      settings: xl_area=[0, 0, 0, 0, 0, 0, 0]  block_version=9.1.01
  Logical : xbsIndex_r4/Logical  logical_function=OR  inputs=4  en=off  latency=0  precision=Full  arith_type=Unsigned  n_bits=16  bin_pt=0  align_bp=on  dbl_ovrd=off  block_type=logical
      settings: block_version=10.1.1
  Mux{,1..3} (4 alike) : xbsIndex_r4/Mux  inputs=2  en=off  latency=1  precision=Full  arith_type="Signed  (2's comp)"  n_bits=8  bin_pt=2  quantization=Truncate  overflow=Wrap  dbl_ovrd=off  block_type=mux
      settings: xl_area=[0, 0, 0, 0, 0, 0, 0]  block_version=9.1.01
  Scale{,1..3} (4 alike) : xbsIndex_r4/Scale  scale_factor=-1  dbl_ovrd=off  block_type=scale
      settings: infoedit=Scales input by a power of two by adjusting the binary point position.<P><P>Hardware notes: In hardware this block costs nothing.  block_version=9.1.01
  convert_of1 : Subsystem  AncestorBlock=casper_library_misc/convert_of  mask(convert_of){bit_width_i=15, binary_point_i=10, bit_width_o=8, binary_point_o=7, latency=2, overflow=Saturate, quantization=Round  (unbiased: +/- Inf)}
      mask prompts: bit_width_i "Bit Width In"; binary_point_i "Binary Point In"; bit_width_o "Bit Width Out"; binary_point_o "Binary Point Out"; overflow "Overflow Behaviour"; quantization "Quantization Behaviour"
      mask help:
      | Converts from one 2's complement bit-width
      | and/or binary point position to another.
      | Includes underflow/overflow indicator.
      mask init:
      | convert_of_init(gcb, ...
      |     'bit_width_i', bit_width_i, ...
      |     'binary_point_i', binary_point_i, ...
      |     'bit_width_o', bit_width_o, ...
      |     'binary_point_o', binary_point_o, ...
      |     'latency', latency, ...
      |     'overflow', overflow, ...
      |     'quantization', quantization);
      settings: AttributesFormatString=[15,10]->[8,7]
      mask StyleString: edit,edit,edit,edit,edit,popup(Wrap|Saturate|Error),popup(Truncate|Round  (unbiased: +/- Inf)|Round  (unbiased: even values))
  convert_of2 : Subsystem  AncestorBlock=casper_library_misc/convert_of  mask(convert_of){bit_width_i=15, binary_point_i=10, bit_width_o=8, binary_point_o=7, latency=2, overflow=Saturate, quantization=Round  (unbiased: +/- Inf)}
      mask prompts: bit_width_i "Bit Width In"; binary_point_i "Binary Point In"; bit_width_o "Bit Width Out"; binary_point_o "Binary Point Out"; overflow "Overflow Behaviour"; quantization "Quantization Behaviour"
      mask help:
      | Converts from one 2's complement bit-width
      | and/or binary point position to another.
      | Includes underflow/overflow indicator.
      mask init: same as fft_test/fft/fft_direct/butterfly1_0/convert_of1
      settings: AttributesFormatString=[15,10]->[8,7]
      mask StyleString: edit,edit,edit,edit,edit,popup(Wrap|Saturate|Error),popup(Truncate|Round  (unbiased: +/- Inf)|Round  (unbiased: even values))
  convert_of3 : Subsystem  AncestorBlock=casper_library_misc/convert_of  mask(convert_of){bit_width_i=15, binary_point_i=10, bit_width_o=8, binary_point_o=7, latency=2, overflow=Saturate, quantization=Round  (unbiased: +/- Inf)}
      mask prompts: bit_width_i "Bit Width In"; binary_point_i "Binary Point In"; bit_width_o "Bit Width Out"; binary_point_o "Binary Point Out"; overflow "Overflow Behaviour"; quantization "Quantization Behaviour"
      mask help:
      | Converts from one 2's complement bit-width
      | and/or binary point position to another.
      | Includes underflow/overflow indicator.
      mask init: same as fft_test/fft/fft_direct/butterfly1_0/convert_of1
      settings: AttributesFormatString=[15,10]->[8,7]
      mask StyleString: edit,edit,edit,edit,edit,popup(Wrap|Saturate|Error),popup(Truncate|Round  (unbiased: +/- Inf)|Round  (unbiased: even values))
  convert_of4 : Subsystem  AncestorBlock=casper_library_misc/convert_of  mask(convert_of){bit_width_i=15, binary_point_i=10, bit_width_o=8, binary_point_o=7, latency=2, overflow=Saturate, quantization=Round  (unbiased: +/- Inf)}
      mask prompts: bit_width_i "Bit Width In"; binary_point_i "Binary Point In"; bit_width_o "Bit Width Out"; binary_point_o "Binary Point Out"; overflow "Overflow Behaviour"; quantization "Quantization Behaviour"
      mask help:
      | Converts from one 2's complement bit-width
      | and/or binary point position to another.
      | Includes underflow/overflow indicator.
      mask init: same as fft_test/fft/fft_direct/butterfly1_0/convert_of1
      settings: AttributesFormatString=[15,10]->[8,7]
      mask StyleString: edit,edit,edit,edit,edit,popup(Wrap|Saturate|Error),popup(Truncate|Round  (unbiased: +/- Inf)|Round  (unbiased: even values))
  ri_to_c : casper_library_misc/ri_to_c  SystemSampleTime=-1
  ri_to_c1 : casper_library_misc/ri_to_c  SystemSampleTime=-1
  twiddle : Subsystem  AncestorBlock=casper_library_ffts_twiddle/twiddle_general_3mult  mask(twiddle_general_3mult){Coeffs=getfield( getfield( get_param( gcb,'UserData' ), 'parameters'),'Coeffs'), StepPeriod=0, coeffs_bram=off, coeff_bit_width=8, input_bit_width=8, add_latency=2, mult_latency=3, bram_latency=1, conv_latency=2, arch=Virtex5, use_hdl=off, use_embedded=on, quantization=Round  (unbiased: +/- Inf), overflow=Saturate}
      mask prompts: Coeffs "Coefficients:"; StepPeriod "Coefficient Step Period (2^?)"; coeffs_bram "Store coefficients in BRAM"; coeff_bit_width "Coefficient Bit Width"; input_bit_width "Input Bit Width"; add_latency "Add Latency"; mult_latency "Mult Latency"; bram_latency "BRAM Latency"; conv_latency "Convert latency"; arch "Architecture"; use_hdl "Use behavioral HDL for multlipliers"; use_embedded "Use embedded multipliers"; quantization "Quantization Behavior"; overflow "Overflow Behavior"
      mask help:
      | Used in biplex pipelined FFT. Takes advantage that
      | (a+bi)(c+di)=(c(a+b)-b(c+d))+i(b(c+d)+a(c-d)) to
      | save on multipliers at expense of adders.
      mask init:
      | twiddle_general_3mult_init(gcb, ... 
      |     'Coeffs', Coeffs, ...
      |     'StepPeriod', StepPeriod, ...
      |     'coeffs_bram', coeffs_bram, ...
      |     'coeff_bit_width', coeff_bit_width, ...
      |     'input_bit_width', input_bit_width, ...
      |     'add_latency', add_latency, ...
      |     'mult_latency', mult_latency, ...
      |     'bram_latency', bram_latency, ...
      |     'conv_latency', conv_latency, ...
      |     'arch', arch, 'use_hdl', use_hdl, ...
      |     'use_embedded', use_embedded, ...
      |     'quantization', quantization, ...
      |     'overflow', overflow)
      settings: AttributesFormatString=|
      | data=(8,7)
      | coeffs=(7,5)
      | Virtex5
      | (Round  (unbiased: +/- Inf),Saturate)
      mask StyleString: edit,edit,checkbox,edit,edit,edit,edit,edit,edit,popup(Virtex2Pro|Virtex5),checkbox,checkbox,popup(Truncate|Round  (unbiased: +/- Inf)|Round  (unbiased: Even Values)),popup(Wrap|Saturate|Error)
      mask CallbackString:
      | ||||||||||use_hdl = get_param(gcb,'use_hdl');
      | visibs = get_param(gcb, 'MaskVisibilities');
      | if( strcmp(use_hdl,'on')),
      |     set_param(gcb, 'use_embedded','off');
      |     visibs{12} = 'off';
      | else,
      |     visibs{12} = 'on';
      | end
      | set_param(gcb, 'MaskVisibilities', visibs);
      | |||
  a+bw : Outport  OutDataType=sfix(16)  OutScaling=2^0
  a-bw : Outport  Port=2  OutDataType=sfix(16)  OutScaling=2^0
  of : Outport  Port=3  OutDataType=sfix(16)  OutScaling=2^0
  sync_out : Outport  Port=4  OutDataType=sfix(16)  OutScaling=2^0
  wires:
  convert_of4/2(of) -> Logical/4
  convert_of3/2(of) -> Logical/3
  convert_of2/2(of) -> Logical/2
  convert_of1/2(of) -> Logical/1
  convert_of4/1(dout) -> ri_to_c1/2
  Mux3/1 -> convert_of4/1(din)
  AddSub3/1 -> Scale3/1, Mux3/2
  Scale3/1 -> Mux3/3
  convert_of3/1(dout) -> ri_to_c1/1
  Mux2/1 -> convert_of3/1(din)
  AddSub2/1 -> Scale2/1, Mux2/2
  Scale2/1 -> Mux2/3
  convert_of2/1(dout) -> ri_to_c/2
  Mux1/1 -> convert_of2/1(din)
  AddSub1/1 -> Scale1/1, Mux1/2
  Scale1/1 -> Mux1/3
  convert_of1/1(dout) -> ri_to_c/1
  Mux/1 -> convert_of1/1(din)
  twiddle/4(bw_im) -> AddSub3/2, AddSub1/2
  twiddle/3(bw_re) -> AddSub2/2, AddSub/2
  twiddle/2(a_im) -> AddSub3/1, AddSub1/1
  twiddle/1(a_re) -> AddSub2/1, AddSub/1
  sync/1 -> twiddle/3(sync)
  b/1 -> twiddle/2(b)
  a/1 -> twiddle/1(a)
  ri_to_c/1 -> a+bw/1
  ri_to_c1/1 -> a-bw/1
  Delay/1 -> sync_out/1
  AddSub/1 -> Mux/2, Scale/1
  shift/1 -> Delay3/1
  Scale/1 -> Mux/3
  Delay3/1 -> Mux3/1, Mux2/1, Mux1/1, Mux/1
  Logical/1 -> of/1
  twiddle/5(sync_out) -> Delay/1
